simulink model "EMT_ML.before_diagnostic_fixes"  (R2024b)
settings: Solver=ode5  StartTime=0.0  StopTime=200  FixedStep=0.002  RelTol=1e-3
model workspace (MAT data in the model file):
  A = 7.3
  B = 2.71
  C0_shift = 200
  C1_shift = 200
  C2_shift = 200
  Cb = 70
  Cd = 0.6
  EMSInputBus : Simulink.Bus (value not decoded)
  Fb_max = 247500
  JA = 0.4
  JB = 0.4
  JZ = 0.4
  Jc1r2 = 0.01
  Jc3r4 = 0.01
  Jc4 = 0.01
  Je = 2.5
  Jh = 0.01
  Jq1 = 0.01
  Jq2 = 0.01
  Jr1 = 0.01
  Jr3s4 = 0.01
  Js123 = 0.01
  L = 4.472
  NE = [1600 1600 1600 1600 1600 1600 1600 1600 1600 1600 1600 1600 ... (840 elements, 30x28)]
  N_Te = 30
  N_ne = 28
  PE = [0 100.366530527 133.710336161 167.221698607 195.706356687 221.845219395 250.497434286 278.144308305 305.288511886 330.086920096 352.87464656 374.489475338 ... (840 elements, 30x28)]
  PN0 = 0
  Pb_epr = [-45 -45 -40 -30 0 30 40 45 45]
  Pb_max = [0 40 45 45 45]
  Pb_min = [-45 -45 -45 -40 0]
  Pe_ass = 230
  Pe_max = 1103
  Peg = [0 100 120 140 160 180 200 220 240 260 280 300 ... (53 elements, 1x53)]
  R_map = [0.09 0.089 0.09 0.091 0.092 0.093 0.094 0.095 0.096 0.097 0.098]
  SF_C0 = 1.5
  SF_C1 = 1.5
  SF_C2 = 1.5
  SF_Z1 = 1.5
  SF_Z2 = 1.5
  SF_ZD = 1.5
  SOC0 = 60
  SOC_epr = [30 31 50 59 60 61 70 79 80]
  SOC_map = [0 10 20 30 40 50 60 70 80 90 100]
  TA_max_map = [588.855 593.803361345 598.83559322 603.953846154 609.160344828 614.457391304 619.847368421 625.332743363 630.916071429 636.6 642.387272727 648.280733945 ... (115 elements, 1x115)]
  TA_min_map = [-588.855 -593.803361345 -598.83559322 -603.953846154 -609.160344828 -614.457391304 -619.847368421 -625.332743363 -630.916071429 -636.6 -642.387272727 -648.280733945 ... (115 elements, 1x115)]
  TAf = 0
  TB_max_map = [588.855 593.803361345 598.83559322 603.953846154 609.160344828 614.457391304 619.847368421 625.332743363 630.916071429 636.6 642.387272727 648.280733945 ... (115 elements, 1x115)]
  TB_min_map = [-588.855 -593.803361345 -598.83559322 -603.953846154 -609.160344828 -614.457391304 -619.847368421 -625.332743363 -630.916071429 -636.6 -642.387272727 -648.280733945 ... (115 elements, 1x115)]
  TBf = 0
  TE = [0 599 798 998 1168 1324 1495 1660 1822 1970 2106 2235 ... (840 elements, 30x28)]
  TS_A = 0.2
  TS_B = 0.2
  TS_C0 = 0.2
  TS_C1 = 0.2
  TS_C2 = 0.2
  TS_Z = 0.2
  TS_Z1 = 0.2
  TS_Z2 = 0.2
  TS_ZD = 0.2
  TZ_max_map = [537.13125 540.509433962 543.930379747 547.394904459 550.903846154 554.458064516 558.058441558 561.705882353 565.401315789 569.145695364 572.94 576.785234899 ... (131 elements, 1x131)]
  TZ_min_map = [-537.13125 -540.509433962 -543.930379747 -547.394904459 -550.903846154 -554.458064516 -558.058441558 -561.705882353 -565.401315789 -569.145695364 -572.94 -576.785234899 ... (131 elements, 1x131)]
  TZf = 0
  T_generator = [0 185 493.333333333 801.666666667 1110 1418.33333333 1726.66666667]
  T_motor = [0 185 493.333333333 801.666666667 1110 1418.33333333 1726.66666667]
  Te_map = [0 599 798 998 1168 1324 1495 1660 1822 1970 2106 2235 ... (30 elements, 1x30)]
  Te_max = 2754
  Te_max_map = [1168 1324 1495 1660 1822 1970 2106 2235 2355 2458 2543 2606 ... (28 elements, 1x28)]
  Te_start = 1600
  Tef = 100
  Teg = [0 596.8125 636.6 718.741935484 799.916230366 859.41 954.422788606 954.9 996.417391304 1078.98305085 1114.05 1169.26530612 ... (53 elements, 1x53)]
  Temax = 998
  Time = [0 0.1 0.2 0.3 0.4 0.5 0.6 0.7 0.8 0.9 1 1.1 ... (2001 elements, 1x2001)]
  Time_ele = [0 4 8 12 16 20 24 28 32 36 40 44 ... (401 elements, 1x401)]
  Time_fg = [0 2 4 6 8 10 12 14 16 18 20 22 ... (801 elements, 1x801)]
  Tmax_C0 = 2754
  Tmax_C1 = 3505.25455609
  Tmax_C2 = 3505.25455609
  Tmax_Z1 = 5584.80955498
  Tmax_Z2 = 16307.6439005
  Tmax_ZD = 3855.6
  Ts_e = 0.1
  Uoc_map = [814.5 917 933.25 945.75 958.25 969.25 978 985.25 993.25 1003.25 1050]
  V_Shift12 = 32
  V_Shift21 = 25
  V_Start = 10
  Voltage0 = 900
  Voltage_epr = [750 760 900 1000 1050]
  Y_engine = 0.955
  Yc = 0.98
  Yh = 0.96
  Yo = 0.92
  Yq = 0.94
  Z1_shift = 200
  Z2_shift = 200
  a11 = 1.54241568346
  a11_L = 1.54241568346
  a12 = -3.86074191629
  a12_L = 2.43173643789
  a21 = -1.04963112005
  a22 = 2.46948356808
  b11 = 0
  b11_L = 0
  b12 = 3.33
  b12_L = 7.8036
  b21 = 2.23571428571
  b22 = -2.13
  c11 = -0.648333656565
  c12 = 0
  c21 = -0.648333656565
  c22 = 0.680511182109
  controller_id = 1
  controller_name = 'Existing heuristic-grid EMS'
  cycle_grade = [0 0 0 0 0 0 0 0 0 0 0 0 ... (2001 elements, 1x2001)]
  cycle_road = [0.045 0.045 0.045 0.045 0.045 0.045 0.045 0.045 0.045 0.045 0.045 0.045 ... (2001 elements, 1x2001)]
  cycle_steering = [0 0 0 0 0 0 0 0 0 0 0 0 ... (2001 elements, 1x2001)]
  cycle_time = [0 0.1 0.2 0.3 0.4 0.5 0.6 0.7 0.8 0.9 1 1.1 ... (2001 elements, 1x2001)]
  d11 = -0.751666343435
  d12 = 0.3003003003
  d21 = -0.751666343435
  d22 = 0.319488817891
  e11 = -1.54241568346
  e12 = 0
  e21 = 1.04963112005
  e22 = -2.23571428571
  eff_generator = [0.8 0.8 0.79 0.79 0.76 0.74 0.72 0.8 0.85 0.88 0.85 0.8 ... (84 elements, 7x12)]
  eff_motor = [0.8 0.8 0.79 0.79 0.76 0.74 0.72 0.8 0.85 0.88 0.85 0.8 ... (84 elements, 7x12)]
  ele_map = [10 11.46 14.13 19.24 20.94 23.21 20.29 20.23 22.28 17.66 16.24 18.95 ... (401 elements, 1x401)]
  ems_runtime_config : object (value not decoded)
  f11 = -3.86074191629
  f12 = 3.33
  f21 = 2.46948356808
  f22 = -2.13
  fg = 0.045
  fg_map = [0.0125 0.0215 0.0332 0.0452 0.0525 0.0589 0.0584 0.0592 0.0621 0.0576 0.055 0.0572 ... (801 elements, 1x801)]
  fuel_gpkwh = [269.874826377 269.874826377 260.084605263 254.895150301 249.802821062 244.062054381 234.972466555 226.630558735 223.93243551 227.612775381 231.379615385 228.983738255 ... (840 elements, 30x28)]
  fuel_map = [269.874826377 269.874826377 260.084605263 254.895150301 249.802821062 244.062054381 234.972466555 226.630558735 223.93243551 227.612775381 231.379615385 228.983738255 ... (840 elements, 30x28)]
  fuel_map_N = [269.874826377 269.874826377 260.084605263 254.895150301 249.802821062 nan nan nan nan nan nan nan ... (840 elements, 30x28)]
  i = 28
  ic = 4.42
  iq = 1.4
  it = 4
  j = 30
  k1 = 2.13
  k2 = 2.13
  k3 = 2.33
  k4 = 1.92
  kh = 2.88
  kq = 2.17
  kt = 1.83
  mass = 45000
  miu_max = 0.8
  nA_map = [-6000 -5950 -5900 -5850 -5800 -5750 -5700 -5650 -5600 -5550 -5500 -5450 ... (115 elements, 1x115)]
  nA_max = 6000
  nA_min = -6000
  nB_map = [-6000 -5950 -5900 -5850 -5800 -5750 -5700 -5650 -5600 -5550 -5500 -5450 ... (115 elements, 1x115)]
  nB_max = 6000
  nB_min = -6000
  nB_start = 0
  nZ_map = [-8000 -7950 -7900 -7850 -7800 -7750 -7700 -7650 -7600 -7550 -7500 -7450 ... (131 elements, 1x131)]
  nZ_max = 8000
  nZ_min = -8000
  n_generator = [0 318.5 796.25 1274 1751.75 2229.5 2707.25 3185 3662.75 4140.5 4618.25 7007]
  n_motor = [0 318.5 796.25 1274 1751.75 2229.5 2707.25 3185 3662.75 4140.5 4618.25 7007]
  ne_idl = 3000
  ne_map = [1600 1700 1800 1900 2000 2100 2200 2300 2400 2500 2600 2700 ... (28 elements, 1x28)]
  ne_max = 4200
  ne_min = 1600
  ne_start = 200
  neg = [1600 1600 1800 1860 1910 2000 2001 2200 2300 2301 2400 2450 ... (53 elements, 1x53)]
  no_Shift12 = 1589.43589002
  no_Shift21 = 1241.74678908
  rz = 0.318
  startup_feedback_delay_s = 0.002
  startup_power_share = 0.5
  startup_speed_regularizer_rpm = 100
  v_cyc = [0 0 0 0 0 0 0 0 0 0 0 0 ... (2001 elements, 1x2001)]
  voltage_HighA = 1050
  voltage_HighB = 1050
  voltage_HighZ = 1050
  voltage_LowA = 750
  voltage_LowB = 750
  voltage_LowZ = 750
symbols that are objects in the model workspace (value not decoded): ems_runtime_config
undefined symbols (not defined in the file or in its folder): sigbuilder_block
libraries: fl_lib x82, nesl_utility x55, simulink x49, sdl_lib x10, simulink_need_slupdate x6, powerlib_extras x1
(part 2 of 7)

== system EMT_ML.before_diagnostic_fixes/Battery ==
  Battery : Subsystem  mask(Battery model){Cb=Cb, SOC0=SOC0, SOC_map=SOC_map, R_map=R_map, Uoc_map=Uoc_map}
      mask prompts: Cb "Capacity (Ah)"; SOC0 "Initial SOC (%)"; SOC_map "State of Charge map (%)"; R_map "Internal resistance map (oms)"; Uoc_map "Open circult voltage map(V)"
      mask help:
      | The length of Open circult voltage map and Internal resistance map is the same with State of Charge map.
      | The power of the battery is positive when it supplies energy, so it's negative when it stores energy.
  Solver Configuration : nesl_utility/Solver Configuration  PhysicalDomain=network_engine_domain  SubClassName=solver  LeftPortType=input  RightPortType=generic  Tones=[]  Harmonics=[]  SimulateNoise=off  Profile=off  UseLocalSampling=off  EnableSwitchedLinearOptims=on  FrequencyDomain=off  UseCCode=off  RelTol=0.001  AbsTol=1e-06  MinStep=1e-09  ToWorkspace=off  RevertToSquareIcSolve=off  NumHomotopyIterations=100  PhasorMode=off  PhasorModeNumHarmonics=1  ConsistencySolver=NEWTON_FTOL  IndexReductionMethod=DerivativeReplacement  DoDC=off  ResidualTolerance=1e-9  ConsistencyTolSource=GLOBAL  ConsistencyAbsTol=0.001  ConsistencyRelTol=0.001  ConsistencyTolFactor=0.001  UseLocalSolver=off  LocalSolverChoice=NE_BACKWARD_EULER_ADVANCER  ResolveIndetEquations=on  FunctionEvalNumThread=1  LocalSolverSampleTime=.001  DoFixedCost=off  MaxNonlinIter=3  MaxModeIter=2  ComputeImpulses=off  ImpulseIterations=2  LinearAlgebra=Sparse  LinearAlgebraNumThread=0  EquationFormulation=NE_TIME_EF  DelaysMemoryBudget=1024  AutomaticFiltering=on  FilteringTimeConstant=0.001  PartitionStorageMethod=AS_NEEDED  PartitionMemoryBudget=1024  PartitionMethod=FAST  MultibodyUseLocalSolver=off  MultibodyLocalSolverChoice=ODE1  MultibodyLocalSolverSampleTime=0.001
  State : Subsystem
  + bat : PMIOPort  Side=Left
  - bat : PMIOPort  Port=2  Side=Left
  wires:
  Battery/1(Voltage) -> State/1(U)
  Battery/2(Current) -> State/2(I)
  Battery/3(SOC) -> State/3(SOC)
  [ElectricPower] -> Battery/1(ElectricPower)
  connections:
  - bat/RConn1 -- Battery/LConn2 -- Solver Configuration/RConn1
  Battery/LConn1 -- + bat/RConn1

== system EMT_ML.before_diagnostic_fixes/Control Unit ==
  Control : Subsystem
  Demux : Demux  Outputs=7
      settings: DisplayOption=none
  Driver : Subsystem
  tag scope: Fb_com=global, Press=global, TA_com=global, TB_com=global, TZ_com=global, Te_com=global, engine_switch=global
  wires:
  Control/1(command) -> Demux/1
  Demux/1 -> [Press]
  Demux/2 -> [engine_switch]
  Demux/3 -> [Te_com]
  Demux/4 -> [TA_com]
  Demux/5 -> [TB_com]
  Demux/6 -> [TZ_com]
  Demux/7 -> [Fb_com]

== system EMT_ML.before_diagnostic_fixes/Front Gear ==
  C0 : Subsystem
  Subsystem : Subsystem
  iq : sdl_lib/Gears/Simple Gear  ratio=iq  rotation_direction=3-2*(1)  friction_model=2  T_noload=0.1 N*m  T_nom=5 N*m  efficiency_nom=0.8  efficiency=Yq  temperature_TLU=[ 280 300 320 ] K  load_TLU=[ 1 5 10 ] N*m  efficiency_TLU=[ 0.95 0.9 0.85 ]  efficiency_TLU2=[ 0.85 0.8 0.75; 0.95 0.9 0.85; 0.85 0.8 0.7 ]  w_thr=0.01 rad/s  pwr_thr=0.001 W  enable_backlash=false  hardstop_model=simscape.enum.hardstop.smooth  backlash_distance=1e-3 mm  r_base=0.1 m  transition=1e-4 mm  backlash_stiffness=1e6 N/m  backlash_damping=1e3 N*s/m  coeff_rest=0.7  v_tol=0.001 m/s  f_tol=0 N  mu_visc=[ 0 0 ] N*m/(rad/s)  thermal_mass=50 J/K  temperature_specify=off  temperature_priority=High  temperature=300 K  temperature_nominal_specify=off  temperature_nominal_value=1  temperature_nominal_unit=K  x_backlash_specify=off  x_backlash_priority=None  x_backlash=0 mm  x_backlash_nominal_specify=off  x_backlash_nominal_value=1  x_backlash_nominal_unit=mm  f_hardstop_specify=off  f_hardstop_priority=None  f_hardstop=0 N  f_hardstop_nominal_specify=off  f_hardstop_nominal_value=1  f_hardstop_nominal_unit=N  v_backlash_specify=off  v_backlash_priority=None  v_backlash=0 m/s  v_backlash_nominal_specify=off  v_backlash_nominal_value=1  v_backlash_nominal_unit=m/s
  In : PMIOPort  Side=Left
  Out : PMIOPort  Port=2  Side=Right
  tag scope: Pi_act=global
  wires:
  Subsystem/1(power) -> [Pi_act]
  connections:
  C0/RConn1 -- iq/LConn1
  Subsystem/RConn1 -- C0/LConn1
  In/RConn1 -- Subsystem/LConn1
  iq/RConn1 -- Out/RConn1

== system EMT_ML.before_diagnostic_fixes/Power Coupler  ==
  C1 : Subsystem
  Z1 : Subsystem
  Z2 : Subsystem
  k1 : sdl_lib/Gears/Planetary Gear  rs_ratio=k1  friction_model=2  efficiency=[ 0.97 0.98 ]  temperature_TLU=[ 280 300 320 ] K  efficiency_sp_TLU=[ 0.95 0.9 0.85 ]  efficiency_rp_TLU=[ 0.95 0.9 0.85 ]  pwr_thr=[ 0.001 0.001 ] W  mu_visc=[ 0 0 ] N*m/(rad/s)  model_inertia=0  sun_inertia=1e-10 kg*m^2  ring_inertia=1e-10 kg*m^2  carrier_inertia=1e-10 kg*m^2  carrier_radius=0.01 m  planet_inertia=0.001 kg*m^2  planet_mass=1e-10 kg  thermal_mass=50 J/K  T_init=300 K
  k2 : sdl_lib/Gears/Planetary Gear  rs_ratio=k2  friction_model=2  efficiency=[ 0.97 0.98 ]  temperature_TLU=[ 280 300 320 ] K  efficiency_sp_TLU=[ 0.95 0.9 0.85 ]  efficiency_rp_TLU=[ 0.95 0.9 0.85 ]  pwr_thr=[ 0.001 0.001 ] W  mu_visc=[ 0 0 ] N*m/(rad/s)  model_inertia=0  sun_inertia=1e-10 kg*m^2  ring_inertia=1e-10 kg*m^2  carrier_inertia=1e-10 kg*m^2  carrier_radius=0.01 m  planet_inertia=0.001 kg*m^2  planet_mass=1e-10 kg  thermal_mass=50 J/K  T_init=300 K
  k3 : sdl_lib/Gears/Planetary Gear  rs_ratio=k3  friction_model=2  efficiency=[ 0.97 0.98 ]  temperature_TLU=[ 280 300 320 ] K  efficiency_sp_TLU=[ 0.95 0.9 0.85 ]  efficiency_rp_TLU=[ 0.95 0.9 0.85 ]  pwr_thr=[ 0.001 0.001 ] W  mu_visc=[ 0 0 ] N*m/(rad/s)  model_inertia=0  sun_inertia=1e-10 kg*m^2  ring_inertia=1e-10 kg*m^2  carrier_inertia=1e-10 kg*m^2  carrier_radius=0.01 m  planet_inertia=0.001 kg*m^2  planet_mass=1e-10 kg  thermal_mass=50 J/K  T_init=300 K
  k4 : sdl_lib/Gears/Planetary Gear  rs_ratio=k4  friction_model=2  efficiency=[ 0.97 0.98 ]  temperature_TLU=[ 280 300 320 ] K  efficiency_sp_TLU=[ 0.95 0.9 0.85 ]  efficiency_rp_TLU=[ 0.95 0.9 0.85 ]  pwr_thr=[ 0.001 0.001 ] W  mu_visc=[ 0 0 ] N*m/(rad/s)  model_inertia=0  sun_inertia=1e-10 kg*m^2  ring_inertia=1e-10 kg*m^2  carrier_inertia=1e-10 kg*m^2  carrier_radius=0.01 m  planet_inertia=0.001 kg*m^2  planet_mass=1e-10 kg  thermal_mass=50 J/K  T_init=300 K
  motor A : PMIOPort  Tag=PMCPort  Side=Left
  motor B : PMIOPort  Tag=PMCPort  Port=2  Side=Right
  lnput : PMIOPort  Tag=PMCPort  Port=3  Side=Left
  output : PMIOPort  Tag=PMCPort  Port=4  Side=Right
  connections:
  k3/RConn2 -- k2/RConn2 -- k1/RConn2 -- motor B/RConn1
  C1/LConn1 -- k1/LConn1 -- k2/RConn1
  k1/RConn1 -- motor A/RConn1
  Z2/LConn1 -- k3/RConn1 -- k4/RConn2
  output/RConn1 -- k3/LConn1 -- C1/RConn1 -- k4/RConn1
  Z1/LConn1 -- k4/LConn1
  lnput/RConn1 -- k2/LConn1

== system EMT_ML.before_diagnostic_fixes/Rear Gear ==
  Rear Gear : Subsystem
  Subsystem : Subsystem
  vehicle : PMIOPort  Side=Right
  output : PMIOPort  Port=2  Side=Left
  tag scope: Po_act=global
  wires:
  Subsystem/1(power) -> [Po_act]
  connections:
  vehicle/RConn1 -- Rear Gear/RConn1
  output/RConn1 -- Subsystem/LConn1
  Subsystem/RConn1 -- Rear Gear/LConn1

== system EMT_ML.before_diagnostic_fixes/Simulation Results ==
  Battery Viewer : Subsystem
      mask Display: disp('Battery')
  Clutch & Brake Viewer : Subsystem
      mask Display: disp('Clutches && Brakes')
  Control Viewer : Subsystem
      mask Display: disp('Control')
  Engine Viewer : Subsystem
      mask Display: disp('Engine')
  Vehicle Viewer : Subsystem
      mask Display: disp('Vehicle')
  motorA Viewer : Subsystem
      mask Display: disp('Motor A')
  motorB Viewer : Subsystem
      mask Display: disp('Motor B')
  motorZ Viewer : Subsystem
      mask Display: disp('Motor Z')

== system EMT_ML.before_diagnostic_fixes/Vehicle dynamics ==
  State : Subsystem
  vehicle dynamic : Subsystem  mask{mass=mass, A=A, rz=rz, L=L, B=B, Cd=Cd, miu_max=miu_max}
      mask prompts: mass "Entire vehicle mass (kg)"; A "Windward area (m^2)"; rz "Radius of the wheel(m)"; L "Length of track (m)"; B "Width of track (m)"; Cd "Drag coefficient"; miu_max "Steering resistance coefficient"
  vehicle : PMIOPort  Side=Left
  wires:
  vehicle dynamic/2(Td_Left) -> State/2(Td_Left)
  vehicle dynamic/1(v_Left) -> State/1(v_Left)
  vehicle dynamic/4(v_Right) -> State/4(v_Right)
  vehicle dynamic/5(Td_rRght) -> State/5(Td_Right)
  [Fb_com] -> vehicle dynamic/1(Fb)
  vehicle dynamic/3(Tf_Left) -> State/3(Tf_Left)
  vehicle dynamic/6(Tf_rRght) -> State/6(Tf_Right)
  [fg_act] -> vehicle dynamic/2(fg)
  [angle] -> vehicle dynamic/3(angle)
  connections:
  vehicle/RConn1 -- vehicle dynamic/LConn1 -- vehicle dynamic/LConn2

== system EMT_ML.before_diagnostic_fixes/engine ==
  Engine : Subsystem  mask(Engine){ne_map=ne_map, Te_max_map=Te_max_map, Tef=Tef, Je=Je, T=Ts_e, Y_engine=Y_engine, P_ass=Pe_ass, Te_start=Te_start}
      mask prompts: ne_map "External characteristic speed (r/min)"; Te_max_map "External characteristic torque(Nm)"; Tef "frictional resistance (Nm)"; Je "rotational inertia(kg/m^2)"; T "First-order delay time  (s)"; Y_engine "Efficinecy of the engine"; P_ass "Power Requriement of auxiliaries (kW)"; Te_start "Engine start torque"
      mask help: Just input the parameters.
  Solver Configuration : nesl_utility/Solver Configuration  PhysicalDomain=network_engine_domain  SubClassName=solver  LeftPortType=input  RightPortType=generic  Tones=[]  Harmonics=[]  SimulateNoise=off  Profile=off  UseLocalSampling=off  EnableSwitchedLinearOptims=on  FrequencyDomain=off  UseCCode=off  RelTol=0.001  AbsTol=1e-06  MinStep=1e-09  ToWorkspace=off  RevertToSquareIcSolve=off  NumHomotopyIterations=100  PhasorMode=off  PhasorModeNumHarmonics=1  ConsistencySolver=NEWTON_FTOL  IndexReductionMethod=DerivativeReplacement  DoDC=off  ResidualTolerance=1e-9  ConsistencyTolSource=GLOBAL  ConsistencyAbsTol=0.001  ConsistencyRelTol=0.001  ConsistencyTolFactor=0.001  UseLocalSolver=off  LocalSolverChoice=NE_BACKWARD_EULER_ADVANCER  ResolveIndetEquations=on  FunctionEvalNumThread=1  LocalSolverSampleTime=.001  DoFixedCost=off  MaxNonlinIter=3  MaxModeIter=2  ComputeImpulses=off  ImpulseIterations=2  LinearAlgebra=Sparse  LinearAlgebraNumThread=0  EquationFormulation=NE_TIME_EF  DelaysMemoryBudget=1024  AutomaticFiltering=on  FilteringTimeConstant=0.001  PartitionStorageMethod=AS_NEEDED  PartitionMemoryBudget=1024  PartitionMethod=FAST  MultibodyUseLocalSolver=off  MultibodyLocalSolverChoice=ODE1  MultibodyLocalSolverSampleTime=0.001
  State : Subsystem
  Connection Port : PMIOPort  Side=Right
  wires:
  Engine/1(ne_act) -> State/1(ne)
  Engine/2(Te_act) -> State/2(Te)
  [engine_switch] -> Engine/2(switch)
  [Te_com] -> Engine/1(Te_com)
  connections:
  Connection Port/RConn1 -- Engine/RConn1 -- Solver Configuration/RConn1

== system EMT_ML.before_diagnostic_fixes/motorA ==
  Motor : Subsystem  mask(Motor){nm_map=nA_map, Tm_max_map=TA_max_map*1.5, Tm_min_map=TA_min_map*1.5, Tmf=TAf, Jm=JA, n_motor=n_motor, T_motor=T_motor, eff_motor=eff_motor, n_generator=n_generator, T_generator=T_generator, eff_generator=eff_generator, T=TS_A}
      mask prompts: nm_map "motor speed map (r/min)"; Tm_max_map "motor max torque map (Nm)"; Tm_min_map "motor min torque map  (Nm)"; Tmf "frictional resistance   (Nm)"; Jm "rotational inertia (km/m^2)"; n_motor "motor speed (r/min)"; T_motor "motor torque (Nm)"; eff_motor "motor efficiency"; n_generator "generator speed (r/min)"; T_generator "generator torque  (Nm)"; eff_generator "generator efficiency"; T "First-order delay time  (s)"
      mask help: The external and efficiency characteristics are needed. When the speed of the motor is too low or too high, it will work at its lowest or highest speed. The influence between voltage and torque is considered.
  State : Subsystem
  Connection Port : PMIOPort  Side=Right
  + mot : PMIOPort  Port=2  Side=Left
  - mot : PMIOPort  Port=3  Side=Left
  wires:
  Motor/4(power_ele) -> State/4(PA)
  Motor/3(voltage) -> State/3(UA)
  Motor/2(Tm_act) -> State/2(TA)
  Motor/1(nm_act) -> State/1(nA)
  [TA_com] -> Motor/1(Tm_com)
  connections:
  - mot/RConn1 -- Motor/LConn2
  + mot/RConn1 -- Motor/LConn1
  Connection Port/RConn1 -- Motor/RConn1

== system EMT_ML.before_diagnostic_fixes/motorB ==
  Motor : Subsystem  mask(Motor){nm_map=nB_map, Tm_max_map=TB_max_map*1.5, Tm_min_map=TB_min_map*1.5, Tmf=TBf, Jm=JB, n_motor=n_motor, T_motor=T_motor, eff_motor=eff_motor, n_generator=n_generator, T_generator=T_generator, eff_generator=eff_generator, T=TS_B}
      mask prompts: nm_map "motor speed map (r/min)"; Tm_max_map "motor max torque map (Nm)"; Tm_min_map "motor min torque map  (Nm)"; Tmf "frictional resistance   (Nm)"; Jm "rotational inertia (km/m^2)"; n_motor "motor speed (r/min)"; T_motor "motor torque (Nm)"; eff_motor "motor efficiency"; n_generator "generator speed (r/min)"; T_generator "generator torque  (Nm)"; eff_generator "generator efficiency"; T "First-order delay time  (s)"
      mask help: The external and efficiency characteristics are needed. When the speed of the motor is too low or too high, it will work at its lowest or highest speed. The influence between voltage and torque is considered.
  State : Subsystem
  Connection Port : PMIOPort  Side=Left
  + mot : PMIOPort  Port=2  Side=Right
  - mot : PMIOPort  Port=3  Side=Right
  wires:
  [TB_com] -> Motor/1(Tm_com)
  Motor/1(nm_act) -> State/1(nB)
  Motor/2(Tm_act) -> State/2(TB)
  Motor/3(voltage) -> State/3(UB)
  Motor/4(power_ele) -> State/4(PB)
  connections:
  Motor/RConn1 -- Connection Port/RConn1
  + mot/RConn1 -- Motor/LConn1
  - mot/RConn1 -- Motor/LConn2

== system EMT_ML.before_diagnostic_fixes/Battery/Battery ==
  ElectricPower : Inport
  1-D Lookup Table : Lookup_n-D  NumberOfTableDimensions=1  BreakpointsForDimension1=SOC_map  Table=Uoc_map  RndMeth=Simplest
  1-D Lookup Table1 : Lookup_n-D  NumberOfTableDimensions=1  BreakpointsForDimension1=SOC_map  Table=R_map  RndMeth=Simplest
  Add1 : Sum
  Controlled Voltage Source : fl_lib/Electrical/Electrical Sources/Controlled Voltage Source
  Current Sensor : fl_lib/Electrical/Electrical Sensors/Current Sensor
  Electrical Reference : fl_lib/Electrical/Electrical Elements/Electrical Reference
  Electronic Equipment : Subsystem
  Memory : Memory  InitialCondition=SOC0
  PS-Simulink Converter1 : nesl_utility/PS-Simulink Converter  PhysicalDomain=network_engine_domain  SubClassName=ps_output  LeftPortType=input  RightPortType=output  PseudoPeriodic=off  Frequencies=[]  VectorFormat=1-D array  Unit=A  AffineConversion=off
  PS-Simulink Converter2 : nesl_utility/PS-Simulink Converter  PhysicalDomain=network_engine_domain  SubClassName=ps_output  LeftPortType=input  RightPortType=output  PseudoPeriodic=off  Frequencies=[]  VectorFormat=1-D array  Unit=V  AffineConversion=off
  SOC Estimation : Subsystem
  Simulink-PS Converter : nesl_utility/Simulink-PS Converter  PhysicalDomain=network_engine_domain  SubClassName=ps_input  LeftPortType=input  RightPortType=output  PseudoPeriodic=off  Frequencies=[]  NoiseDistribution=none  NoiseParameters=[]  Unit=V  AffineConversion=off  FilteringAndDerivatives=filter  SimscapeFilterOrder=1  InputFilterTimeConstant=.001  UdotUserProvided=1
  Simulink-PS Converter1 : nesl_utility/Simulink-PS Converter  PhysicalDomain=network_engine_domain  SubClassName=ps_input  LeftPortType=input  RightPortType=output  PseudoPeriodic=off  Frequencies=[]  NoiseDistribution=none  NoiseParameters=[]  Unit=Ohm  AffineConversion=off  FilteringAndDerivatives=filter  SimscapeFilterOrder=1  InputFilterTimeConstant=.001  UdotUserProvided=1
  Variable Resistor : fl_lib/Electrical/Electrical Elements/Variable Resistor  Rmin=0.1 Ohm  thermalEnable=false  thermal_mass=1 J/K  i_specify=off  i_priority=None  i=0 A  i_nominal_specify=off  i_nominal_value=1  i_nominal_unit=A  v_specify=off  v_priority=None  v=0 V  v_nominal_specify=off  v_nominal_value=1  v_nominal_unit=V  T_specify=off  T_priority=None  T=300 K  T_nominal_specify=off  T_nominal_value=1  T_nominal_unit=K
  Voltage Sensor : fl_lib/Electrical/Electrical Sensors/Voltage Sensor
  pumb : Constant  Value=14
  + : PMIOPort  Side=Left
  - : PMIOPort  Port=2  Side=Left
  Voltage : Outport
  Current : Outport  Port=2
  SOC : Outport  Port=3
  wires:
  Memory/1 -> 1-D Lookup Table1/1, 1-D Lookup Table/1
  1-D Lookup Table1/1 -> Simulink-PS Converter1/1
  1-D Lookup Table/1 -> Simulink-PS Converter/1
  SOC Estimation/1(SOC) -> Memory/1, SOC/1
  PS-Simulink Converter1/1 -> SOC Estimation/1(I), Current/1
  PS-Simulink Converter2/1 -> Voltage/1
  Add1/1 -> Electronic Equipment/1(power)
  ElectricPower/1 -> Add1/2
  pumb/1 -> Add1/1
  connections:
  Simulink-PS Converter1/RConn1 -- Variable Resistor/LConn1
  Controlled Voltage Source/RConn1 -- Simulink-PS Converter/RConn1
  Current Sensor/RConn1 -- PS-Simulink Converter1/LConn1
  PS-Simulink Converter2/LConn1 -- Voltage Sensor/RConn1
  Electronic Equipment/RConn2 -- Variable Resistor/RConn1 -- Voltage Sensor/RConn2 -- -/RConn1
  Electronic Equipment/RConn1 -- +/RConn1 -- Voltage Sensor/LConn1 -- Current Sensor/RConn2
  Controlled Voltage Source/RConn2 -- Variable Resistor/LConn2 -- Electrical Reference/LConn1
  Current Sensor/LConn1 -- Controlled Voltage Source/LConn1

== system EMT_ML.before_diagnostic_fixes/Battery/State ==
  U : Inport
  I : Inport  Port=2
  SOC : Inport  Port=3
  Gain : Gain  Gain=1/1000
  Product : Product  RndMeth=Zero
  tag scope: Current=global, Pb_act=global, SOC=global, Voltage=global
  wires:
  SOC/1 -> [SOC]
  I/1 -> [Current], Product/2
  U/1 -> [Voltage], Product/1
  Gain/1 -> [Pb_act]
  Product/1 -> Gain/1

== system EMT_ML.before_diagnostic_fixes/Control Unit/Control ==
  EVT1_H Stage : Subsystem
  EVT2 Stage : Subsystem
  Multiport Switch : MultiPortSwitch  DataPortOrder=Zero-based contiguous  Inputs=4  DiagnosticForDefault=None  zeroidx=on  SaturateOnIntegerOverflow=off  InputSameDT=off
  Power Distribution : Subsystem
  Prepare Stage : Subsystem
  Shift Stage : Subsystem
  Stage Judge : Subsystem
  command : Outport
  wires:
  EVT2 Stage/1(control) -> Multiport Switch/5
  Shift Stage/1(control) -> Multiport Switch/4
  EVT1_H Stage/1(control) -> Multiport Switch/3
  Prepare Stage/1(control) -> Multiport Switch/2
  Stage Judge/1(stage) -> Multiport Switch/1
  Multiport Switch/1 -> command/1

== system EMT_ML.before_diagnostic_fixes/Control Unit/Driver ==
  Electric Power Requirement : Subsystem
      mask Display: image(imread('Electric Equiments.jpg'))
  Gears : Subsystem
      mask Display: image(imread('gears.jpg'))
  Grade Angle : Subsystem
      mask Display: image(imread('Grade.jpg'))
  Ground Resistance Coefficient : Subsystem
      mask Display: image(imread('Ground.jpg'))
  "Pedal " : Subsystem
      mask Display: image(imread('pedal.jpg'))
  Wheel Angle : Subsystem
      mask Display: image(imread('Wheel.jpg'))

== system EMT_ML.before_diagnostic_fixes/Front Gear/C0 ==
  Abs : Abs  SaturateOnIntegerOverflow=off
  Add : Sum  Inputs=+-
  C0 : Subsystem
  Power : Subsystem
  Power1 : Subsystem
  In : PMIOPort  Side=Left
  Out : PMIOPort  Port=2  Side=Right
  tag scope: C0_loss=global, C0_rela=global
  wires:
  [Press_C0] -> C0/1(Press)
  C0/1(r/min) -> [C0_rela]
  Power1/1(kW) -> Add/2
  Power/1(kW) -> Add/1
  Add/1 -> Abs/1
  Abs/1 -> [C0_loss]
  connections:
  In/RConn1 -- Power/LConn1
  C0/LConn1 -- Power/RConn1
  C0/RConn1 -- Power1/LConn1
  Power1/RConn1 -- Out/RConn1

== system EMT_ML.before_diagnostic_fixes/Front Gear/Subsystem ==
  Gain1 : Gain  Gain=1/9549
  Product3 : Product  RndMeth=Zero
  Speed Sensor : Subsystem  mask(Speed Sensor){}
      mask help: The speed unit is r/min.
  Torque Sensor : Subsystem  mask(Torque Sensor){}
      mask help: The torque unit is Nm.
  in : PMIOPort  Side=Left
  out : PMIOPort  Port=2  Side=Right
  power : Outport
  wires:
  Gain1/1 -> power/1
  Product3/1 -> Gain1/1
  Torque Sensor/1(Nm) -> Product3/2
  Speed Sensor/1(r/min) -> Product3/1
  connections:
  out/RConn1 -- Torque Sensor/RConn1
  Speed Sensor/LConn1 -- Torque Sensor/LConn1 -- in/RConn1

== system EMT_ML.before_diagnostic_fixes/Power Coupler /C1 ==
  Abs : Abs  SaturateOnIntegerOverflow=off
  Add : Sum  Inputs=+-
  C2 : Subsystem
  Power : Subsystem
  Power1 : Subsystem
  In : PMIOPort  Side=Left
  Out : PMIOPort  Port=2  Side=Right
  tag scope: C1_loss=global, C1_rela=global
  wires:
  C2/1(r/min) -> [C1_rela]
  [Press_C1] -> C2/1(Press)
  Add/1 -> Abs/1
  Abs/1 -> [C1_loss]
  Power1/1(kW) -> Add/2
  Power/1(kW) -> Add/1
  connections:
  In/RConn1 -- Power/LConn1
  Power/RConn1 -- C2/LConn1
  C2/RConn1 -- Power1/LConn1
  Power1/RConn1 -- Out/RConn1

== system EMT_ML.before_diagnostic_fixes/Power Coupler /Z1 ==
  Mechanical Rotational Reference : fl_lib/Mechanical/Rotational Elements/Mechanical Rotational Reference
  Z : Subsystem
  Z1 : PMIOPort  Side=Left
  connections:
  Mechanical Rotational Reference/LConn1 -- Z/RConn1
  Z1/RConn1 -- Z/LConn1

== system EMT_ML.before_diagnostic_fixes/Power Coupler /Z2 ==
  Mechanical Rotational Reference : fl_lib/Mechanical/Rotational Elements/Mechanical Rotational Reference
  Z : Subsystem
  Z2 : PMIOPort  Side=Left
  connections:
  Z/LConn1 -- Z2/RConn1
  Mechanical Rotational Reference/LConn1 -- Z/RConn1

== system EMT_ML.before_diagnostic_fixes/Rear Gear/Rear Gear ==
  Inertia : fl_lib/Mechanical/Rotational Elements/Inertia  inertia=Jh/2 kg*m^2  num_ports=foundation.enum.numPorts2.one  w_specify=on  w_priority=High  w=0 rad/s  w_nominal_specify=off  w_nominal_value=1  w_nominal_unit=rad/s  t_specify=off  t_priority=None  t=0 N*m  t_nominal_specify=off  t_nominal_value=1  t_nominal_unit=N*m
  Inertia1 : fl_lib/Mechanical/Rotational Elements/Inertia  inertia=Jc3r4/2 kg*m^2  num_ports=foundation.enum.numPorts2.one  w_specify=on  w_priority=High  w=0 rad/s  w_nominal_specify=off  w_nominal_value=1  w_nominal_unit=rad/s  t_specify=off  t_priority=None  t=0 N*m  t_nominal_specify=off  t_nominal_value=1  t_nominal_unit=N*m
  Simple Gear : sdl_lib/Gears/Simple Gear  ratio=ic*(1+kh)/kh  rotation_direction=3-2*(1)  friction_model=2  T_noload=0.1 N*m  T_nom=5 N*m  efficiency_nom=0.8  efficiency=Yh*Yc  temperature_TLU=[ 280 300 320 ] K  load_TLU=[ 1 5 10 ] N*m  efficiency_TLU=[ 0.95 0.9 0.85 ]  efficiency_TLU2=[ 0.85 0.8 0.75; 0.95 0.9 0.85; 0.85 0.8 0.7 ]  w_thr=0.01 rad/s  pwr_thr=0.001 W  enable_backlash=false  hardstop_model=simscape.enum.hardstop.smooth  backlash_distance=1e-3 mm  r_base=0.1 m  transition=1e-4 mm  backlash_stiffness=1e6 N/m  backlash_damping=1e3 N*s/m  coeff_rest=0.7  v_tol=0.001 m/s  f_tol=0 N  mu_visc=[ 0 0 ] N*m/(rad/s)  thermal_mass=50 J/K  temperature_specify=off  temperature_priority=High  temperature=300 K  temperature_nominal_specify=off  temperature_nominal_value=1  temperature_nominal_unit=K  x_backlash_specify=off  x_backlash_priority=None  x_backlash=0 mm  x_backlash_nominal_specify=off  x_backlash_nominal_value=1  x_backlash_nominal_unit=mm  f_hardstop_specify=off  f_hardstop_priority=None  f_hardstop=0 N  f_hardstop_nominal_specify=off  f_hardstop_nominal_value=1  f_hardstop_nominal_unit=N  v_backlash_specify=off  v_backlash_priority=None  v_backlash=0 m/s  v_backlash_nominal_specify=off  v_backlash_nominal_value=1  v_backlash_nominal_unit=m/s
  In : PMIOPort  Side=Left
  Out : PMIOPort  Port=2  Side=Right
  connections:
  Simple Gear/RConn1 -- Inertia/LConn1 -- Out/RConn1
  Simple Gear/LConn1 -- In/RConn1 -- Inertia1/LConn1

== system EMT_ML.before_diagnostic_fixes/Rear Gear/Subsystem ==
  Gain1 : Gain  Gain=1/9549
  Product3 : Product  RndMeth=Zero
  Speed Sensor : Subsystem  mask(Speed Sensor){}
      mask help: The speed unit is r/min.
  Torque Sensor : Subsystem  mask(Torque Sensor){}
      mask help: The torque unit is Nm.
  in : PMIOPort  Side=Left
  out : PMIOPort  Port=2  Side=Right
  power : Outport
  wires:
  Gain1/1 -> power/1
  Product3/1 -> Gain1/1
  Torque Sensor/1(Nm) -> Product3/2
  Speed Sensor/1(r/min) -> Product3/1
  connections:
  out/RConn1 -- Torque Sensor/RConn1
  Torque Sensor/LConn1 -- in/RConn1 -- Speed Sensor/LConn1

== system EMT_ML.before_diagnostic_fixes/Simulation Results/Battery Viewer ==
  Scope10 : Scope  NumInputPorts=4
  Scope2 : Scope  NumInputPorts=3
  wires:
  [SOC] -> Scope10/1
  [Current] -> Scope10/2
  [Voltage] -> Scope10/3
  [Pb_act] -> Scope10/4
  [PN_com] -> Scope2/1
  [PN_max] -> Scope2/2
  [PN_min] -> Scope2/3

== system EMT_ML.before_diagnostic_fixes/Simulation Results/Clutch & Brake Viewer ==
  Scope6 : Scope  NumInputPorts=4
  Scope7 : Scope  NumInputPorts=4
  Scope8 : Scope  NumInputPorts=4
  wires:
  [Z2_loss] -> Scope8/4
  [Z1_loss] -> Scope8/3
  [C1_loss] -> Scope8/2
  [C0_loss] -> Scope8/1
  [Z2_rela] -> Scope6/4
  [Z1_rela] -> Scope6/3
  [C1_rela] -> Scope6/2
  [C0_rela] -> Scope6/1
  [Press_Z2] -> Scope7/4
  [Press_Z1] -> Scope7/3
  [Press_C1] -> Scope7/2
  [Press_C0] -> Scope7/1

== system EMT_ML.before_diagnostic_fixes/Simulation Results/Control Viewer ==
  Scope{,1,3..4,7} (5 alike) : Scope
  Scope11 : Scope  NumInputPorts=4
  Scope2 : Scope  NumInputPorts=3
  wires:
  [Wheel] -> Scope11/4
  [angle] -> Scope11/3
  [ElectricPower] -> Scope11/2
  [fg_act] -> Scope11/1
  [stage] -> Scope2/1
  [Acc_pedal] -> Scope2/2
  [Dec_pedal] -> Scope2/3
  [Gear] -> Scope1/1
  [mode] -> Scope3/1
  [ZD_Gear] -> Scope/1
  [Wheel] -> Scope7/1
  [ElectricPower] -> Scope4/1

== system EMT_ML.before_diagnostic_fixes/Simulation Results/Engine Viewer ==
  "Fuel " : Subsystem
  Scope1 : Scope  NumInputPorts=4
  Scope12 : Scope  NumInputPorts=2
  Scope2 : Scope  NumInputPorts=3
  Scope4 : Scope  NumInputPorts=2
  Scope5 : Scope  NumInputPorts=2
  wires:
  "Fuel "/2(gpkWh) -> Scope12/2
  "Fuel "/1(fuel_L) -> Scope12/1
  [ne_act] -> Scope1/2
  [Te_act] -> Scope1/3
  [engine_switch] -> Scope1/1
  [Pe_act] -> Scope1/4
  [Pe_act] -> Scope4/2
  [Pe_com] -> Scope4/1
  [ne_act] -> Scope5/2
  [ne_ref] -> Scope5/1
  [Te_act] -> Scope2/3
  [Te_com] -> Scope2/2
  [Te_ref] -> Scope2/1

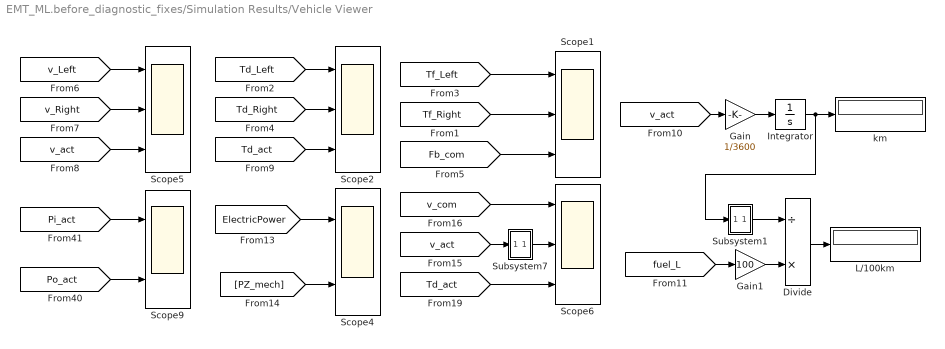
== system EMT_ML.before_diagnostic_fixes/Simulation Results/Vehicle Viewer ==
  Divide : Product  Inputs=/*
  Gain : Gain  Gain=1/3600
  Gain1 : Gain  Gain=100
  Integrator : Integrator
  L/100km : Display
  Scope{1..2,5..6} (4 alike) : Scope  NumInputPorts=3
  Scope4 : Scope  NumInputPorts=2
  Scope9 : Scope  NumInputPorts=2
  Subsystem1 : Subsystem
  Subsystem7 : Subsystem
  km : Display
  wires:
  [Pi_act] -> Scope9/1
  [Po_act] -> Scope9/2
  [v_com] -> Scope6/1
  [v_act] -> Subsystem7/1(0)
  [Td_act] -> Scope6/3
  Subsystem7/1(1) -> Scope6/2
  [v_Left] -> Scope5/1
  [v_Right] -> Scope5/2
  [v_act] -> Scope5/3
  [Td_Right] -> Scope2/2
  [Td_Left] -> Scope2/1
  [Tf_Right] -> Scope1/2
  [Tf_Left] -> Scope1/1
  [Fb_com] -> Scope1/3
  [ElectricPower] -> Scope4/1
  [PZ_mech] -> Scope4/2
  [Td_act] -> Scope2/3
  [v_act] -> Gain/1
  Integrator/1 -> km/1, Subsystem1/1(0)
  Gain/1 -> Integrator/1
  [fuel_L] -> Gain1/1
  Gain1/1 -> Divide/2
  Divide/1 -> L/100km/1
  Subsystem1/1(1) -> Divide/1

== system EMT_ML.before_diagnostic_fixes/Simulation Results/motorA Viewer ==
  Mux : Mux  Inputs=2
  Scope1 : Scope  NumInputPorts=4
  Scope2 : Scope  NumInputPorts=3
  Scope3 : Scope
  Scope4 : Scope
  wires:
  [nA_act] -> Scope1/1
  [TA_act] -> Scope1/2
  [PA_mech] -> Scope1/3
  [PA_ele] -> Scope1/4
  [PA_ele] -> Mux/2
  [PA_mech] -> Mux/1
  Mux/1 -> Scope4/1
  [voltageA] -> Scope3/1
  [TA_act] -> Scope2/3
  [TA_com] -> Scope2/2
  [TA_ref] -> Scope2/1

== system EMT_ML.before_diagnostic_fixes/Simulation Results/motorB Viewer ==
  Mux : Mux  Inputs=2
  Scope1 : Scope  NumInputPorts=4
  Scope2 : Scope  NumInputPorts=3
  Scope3 : Scope
  Scope4 : Scope
  wires:
  [PB_ele] -> Scope1/4
  [TB_act] -> Scope1/2
  [nB_act] -> Scope1/1
  [PB_mech] -> Scope1/3
  [voltageB] -> Scope3/1
  Mux/1 -> Scope4/1
  [PB_mech] -> Mux/1
  [PB_ele] -> Mux/2
  [TB_act] -> Scope2/3
  [TB_com] -> Scope2/2
  [TB_ref] -> Scope2/1

== system EMT_ML.before_diagnostic_fixes/Simulation Results/motorZ Viewer ==
  Mux : Mux  Inputs=2
  Mux1 : Mux  Inputs=2
  Scope1 : Scope  NumInputPorts=3
  Scope2 : Scope  NumInputPorts=3
  Scope3 : Scope
  Scope4 : Scope
  Scope5 : Scope  NumInputPorts=2
  Scope6 : Scope
  wires:
  [PZ_mech] -> Scope1/3
  [TZ_ref] -> Scope2/1
  [TZ_com] -> Scope2/2
  [TZ_act] -> Scope2/3
  [PZ_ele] -> Mux/2
  [PZ_mech] -> Mux/1
  Mux/1 -> Scope4/1
  [voltageZ] -> Scope3/1
  [TZ_act] -> Scope1/2
  [nZ_act] -> Scope1/1
  [nZ_ref] -> Scope5/1
  [nZ_act] -> Scope5/2
  [PZ_com] -> Mux1/2
  [PZ_ref] -> Mux1/1
  Mux1/1 -> Scope6/1

== system EMT_ML.before_diagnostic_fixes/Vehicle dynamics/State ==
  v_Left : Inport
  Td_Left : Inport  Port=2
  Tf_Left : Inport  Port=3
  v_Right : Inport  Port=4
  Td_Right : Inport  Port=5
  Tf_Right : Inport  Port=6
  Sum1 : Sum
  Sum2 : Sum
  Sum3 : Sum
  Tire Radius4 : Gain  Gain=0.5
  tag scope: Td_Left=global, Td_Right=global, Td_act=global, Tf_Left=global, Tf_Right=global, Tf_act=global, v_Left=global, v_Right=global, v_act=global
  wires:
  Td_Left/1 -> [Td_Left], Sum2/1
  v_Left/1 -> [v_Left], Sum1/1
  v_Right/1 -> [v_Right], Sum1/2
  Td_Right/1 -> [Td_Right], Sum2/2
  Sum1/1 -> Tire Radius4/1
  Sum2/1 -> [Td_act]
  Tire Radius4/1 -> [v_act]
  Tf_Left/1 -> Sum3/1, [Tf_Left]
  Tf_Right/1 -> Sum3/2, [Tf_Right]
  Sum3/1 -> [Tf_act]

== system EMT_ML.before_diagnostic_fixes/Vehicle dynamics/vehicle dynamic ==
  Fb : Inport
  fg : Inport  Port=2
  angle : Inport  Port=3
  Fb1 : InportShadow
  angle1 : InportShadow  Port=3
  fg1 : InportShadow  Port=2
  vehicle dynamic : Subsystem
  vehicle dynamic1 : Subsystem
  Left : PMIOPort  Side=Left
  Right : PMIOPort  Port=2  Side=Left
  v_Left : Outport
  Td_Left : Outport  Port=2
  Tf_Left : Outport  Port=3
  v_Right : Outport  Port=4
  Td_rRght : Outport  Port=5
  Tf_rRght : Outport  Port=6
  wires:
  Fb/1 -> vehicle dynamic/1(brake force)
  vehicle dynamic/1(vehicle speed) -> v_Left/1
  vehicle dynamic/2(Driving Torque) -> Td_Left/1
  vehicle dynamic1/1(vehicle speed) -> v_Right/1
  vehicle dynamic1/2(Driving Torque) -> Td_rRght/1
  vehicle dynamic/3(Tf) -> Tf_Left/1
  vehicle dynamic1/3(Tf) -> Tf_rRght/1
  fg/1 -> vehicle dynamic/2(fg)
  angle/1 -> vehicle dynamic/3(angle)
  Fb1/1 -> vehicle dynamic1/1(brake force)
  fg1/1 -> vehicle dynamic1/2(fg)
  angle1/1 -> vehicle dynamic1/3(angle)
  connections:
  Left/RConn1 -- vehicle dynamic/LConn1
  Right/RConn1 -- vehicle dynamic1/LConn1

== system EMT_ML.before_diagnostic_fixes/engine/Engine ==
  Te_com : Inport
  switch : Inport  Port=2
  Inertia1 : fl_lib/Mechanical/Rotational Elements/Inertia  inertia=Je kg*m^2  num_ports=foundation.enum.numPorts2.one  w_specify=on  w_priority=High  w=0 rpm  w_nominal_specify=off  w_nominal_value=1  w_nominal_unit=rad/s  t_specify=off  t_priority=None  t=0 N*m  t_nominal_specify=off  t_nominal_value=1  t_nominal_unit=N*m
  Memory2 : Memory
  Memory3 : Memory
  Speed Sensor : Subsystem  mask(Speed Sensor){}
      mask help: The speed unit is r/min.
  Subsystem : Subsystem
  Subsystem1 : Subsystem
  Torque Actuator : Subsystem  mask(Torque Actuator){}
      mask help: The torque unit is Nm.
  Out : PMIOPort  Side=Right
  ne_act : Outport
  Te_act : Outport  Port=2
  wires:
  Te_com/1 -> Subsystem/2(Te_com)
  Subsystem/2(Torque) -> Torque Actuator/1(torque)
  switch/1 -> Subsystem/3(switch)
  Memory3/1 -> Subsystem/1(ne_act)
  Speed Sensor/1(r/min) -> ne_act/1, Memory3/1, Memory2/1
  Memory2/1 -> Subsystem1/1(ne)
  Subsystem/1(Te_act) -> Te_act/1
  connections:
  Out/RConn1 -- Speed Sensor/LConn1 -- Subsystem1/RConn1 -- Torque Actuator/RConn1 -- Inertia1/LConn1

== system EMT_ML.before_diagnostic_fixes/engine/State ==
  ne : Inport
  Te : Inport  Port=2
  Gain : Gain  Gain=1/9549
  Product : Product  RndMeth=Zero
  tag scope: Pe_act=global, Te_act=global, ne_act=global
  wires:
  ne/1 -> [ne_act], Product/1
  Te/1 -> [Te_act], Product/2
  Product/1 -> Gain/1
  Gain/1 -> [Pe_act]

== system EMT_ML.before_diagnostic_fixes/motorA/Motor ==
  Tm_com : Inport
  Efficiency : Subsystem
  Electrical System : Subsystem
  Mechanical Body : Subsystem
  output : PMIOPort  Side=Right
  + mot : PMIOPort  Port=2  Side=Left
  - mot : PMIOPort  Port=3  Side=Left
  nm_act : Outport
  Tm_act : Outport  Port=2
  voltage : Outport  Port=3
  power_ele : Outport  Port=4
  wires:
  Efficiency/1(power) -> power_ele/1, Electrical System/1(power)
  Tm_com/1 -> Mechanical Body/1(Tm_com)
  Mechanical Body/2(torque) -> Efficiency/2(torque), Tm_act/1
  Mechanical Body/1(speed) -> Efficiency/1(speed), nm_act/1
  Electrical System/1(voltage) -> voltage/1
  connections:
  - mot/RConn1 -- Electrical System/RConn2
  + mot/RConn1 -- Electrical System/RConn1
  output/RConn1 -- Mechanical Body/RConn1

== system EMT_ML.before_diagnostic_fixes/motorA/State ==
  nA : Inport
  TA : Inport  Port=2
  UA : Inport  Port=3
  PA : Inport  Port=4
  Gain : Gain  Gain=1/9549
  Product : Product  RndMeth=Zero
  tag scope: PA_ele=global, PA_mech=global, TA_act=global, nA_act=global, voltageA=global
  wires:
  nA/1 -> [nA_act], Product/1
  TA/1 -> [TA_act], Product/2
  UA/1 -> [voltageA]
  PA/1 -> [PA_ele]
  Product/1 -> Gain/1
  Gain/1 -> [PA_mech]

== system EMT_ML.before_diagnostic_fixes/motorB/Motor ==
  Tm_com : Inport
  Efficiency : Subsystem
  Electrical System : Subsystem
  Mechanical Body : Subsystem
  output : PMIOPort  Side=Right
  + mot : PMIOPort  Port=2  Side=Left
  - mot : PMIOPort  Port=3  Side=Left
  nm_act : Outport
  Tm_act : Outport  Port=2
  voltage : Outport  Port=3
  power_ele : Outport  Port=4
  wires:
  Efficiency/1(power) -> power_ele/1, Electrical System/1(power)
  Tm_com/1 -> Mechanical Body/1(Tm_com)
  Mechanical Body/2(torque) -> Efficiency/2(torque), Tm_act/1
  Mechanical Body/1(speed) -> Efficiency/1(speed), nm_act/1
  Electrical System/1(voltage) -> voltage/1
  connections:
  - mot/RConn1 -- Electrical System/RConn2
  + mot/RConn1 -- Electrical System/RConn1
  output/RConn1 -- Mechanical Body/RConn1

== system EMT_ML.before_diagnostic_fixes/motorB/State ==
  nB : Inport
  TB : Inport  Port=2
  UB : Inport  Port=3
  PB : Inport  Port=4
  Gain : Gain  Gain=1/9549
  Product : Product  RndMeth=Zero
  tag scope: PB_ele=global, PB_mech=global, TB_act=global, nB_act=global, voltageB=global
  wires:
  TB/1 -> [TB_act], Product/2
  UB/1 -> [voltageB]
  PB/1 -> [PB_ele]
  Product/1 -> Gain/1
  Gain/1 -> [PB_mech]
  nB/1 -> [nB_act], Product/1

== system EMT_ML.before_diagnostic_fixes/Battery/Battery/Electronic Equipment ==
  power : Inport
  Constant3 : Constant  Value=interp1(SOC_map,Uoc_map,SOC0)
  Controlled Current Source1 : fl_lib/Electrical/Electrical Sources/Controlled Current Source
  Divie1 : Product  Inputs=*/
  Gain : Gain  Gain=-1000
  Memory2 : Memory  InitialCondition=interp1(SOC_map,Uoc_map,SOC0)
  PS-Simulink Converter : nesl_utility/PS-Simulink Converter  PhysicalDomain=network_engine_domain  SubClassName=ps_output  LeftPortType=input  RightPortType=output  PseudoPeriodic=off  Frequencies=[]  VectorFormat=1-D array  Unit=V  AffineConversion=off
  Simulink-PS Converter : nesl_utility/Simulink-PS Converter  PhysicalDomain=network_engine_domain  SubClassName=ps_input  LeftPortType=input  RightPortType=output  PseudoPeriodic=off  Frequencies=[]  NoiseDistribution=none  NoiseParameters=[]  Unit=A  AffineConversion=off  FilteringAndDerivatives=filter  SimscapeFilterOrder=1  InputFilterTimeConstant=.001  UdotUserProvided=1
  Switch : Switch  Criteria=u2 ~= 0  SaturateOnIntegerOverflow=off  InputSameDT=off
  Voltage Sensor : fl_lib/Electrical/Electrical Sensors/Voltage Sensor
  +ele : PMIOPort  Side=Right
  - ele : PMIOPort  Port=2  Side=Right
  wires:
  Gain/1 -> Simulink-PS Converter/1
  Memory2/1 -> Switch/1, Switch/2
  Switch/1 -> Divie1/2
  Constant3/1 -> Switch/3
  PS-Simulink Converter/1 -> Memory2/1
  Divie1/1 -> Gain/1
  power/1 -> Divie1/1
  connections:
  PS-Simulink Converter/LConn1 -- Voltage Sensor/RConn1
  Voltage Sensor/LConn1 -- Controlled Current Source1/LConn1 -- +ele/RConn1
  Voltage Sensor/RConn2 -- Controlled Current Source1/RConn2 -- - ele/RConn1
  Simulink-PS Converter/RConn1 -- Controlled Current Source1/RConn1

== system EMT_ML.before_diagnostic_fixes/Battery/Battery/SOC Estimation ==
  I : Inport
  Add1 : Sum
  Constant2 : Constant  Value=Cb
  Constant3 : Constant  Value=SOC0
  Divide : Product  Inputs=*/
  Gain : Gain  Gain=-1/36
  Integrator : Integrator
  SOC : Outport
  wires:
  Gain/1 -> Add1/2
  I/1 -> Divide/1
  Add1/1 -> SOC/1
  Constant3/1 -> Add1/1
  Integrator/1 -> Gain/1
  Divide/1 -> Integrator/1
  Constant2/1 -> Divide/2

== system EMT_ML.before_diagnostic_fixes/Control Unit/Control/EVT1_H Stage ==
  Mux : Mux  Inputs=7
  brack force : Subsystem
  clutches condition : Subsystem
  engine swich : Subsystem
  engine torque : Subsystem
  motorA torque : Subsystem
  motorB torque : Subsystem
  motorZ torque : Subsystem
  control : Outport
  wires:
  motorB torque/1(TB_com) -> Mux/5
  motorA torque/1(TA_com) -> Mux/4
  clutches condition/1(clutch_com) -> Mux/1
  engine swich/1(engine_swich) -> Mux/2
  engine torque/1(Te_com) -> Mux/3
  Mux/1 -> control/1
  motorZ torque/1(TZ_com) -> Mux/6
  brack force/1(Fb_com) -> Mux/7

== system EMT_ML.before_diagnostic_fixes/Control Unit/Control/EVT2 Stage ==
  Mux : Mux  Inputs=7
  brack force : Subsystem
  clutches condition : Subsystem
  engine swich : Subsystem
  engine torque : Subsystem
  motorA torque : Subsystem
  motorB torque : Subsystem
  motorZ torque : Subsystem
  control : Outport
  wires:
  motorB torque/1(TB_com) -> Mux/5
  motorA torque/1(TA_com) -> Mux/4
  engine torque/1(Te_com) -> Mux/3
  clutches condition/1(clutch_com) -> Mux/1
  engine swich/1(engine_swich) -> Mux/2
  Mux/1 -> control/1
  brack force/1(Fb_com) -> Mux/7
  motorZ torque/1(TZ_com) -> Mux/6

== system EMT_ML.before_diagnostic_fixes/Control Unit/Control/Power Distribution ==
  Electric Power Requirement : Subsystem
  Feasible Control Range : Subsystem  SystemSampleTime=0.02
  Oil Control : Subsystem
  Optimal Power Distribution : Subsystem  SystemSampleTime=10
  Pedal Interpretation : Subsystem
  Subsystem : Subsystem
  tag scope: Fb_ref=global, TA_ref=global, TB_ref=global, Te_ref=global, ne_ref=global
  wires:
  Feasible Control Range/6(TB_k) -> Optimal Power Distribution/8(TB_k)
  Feasible Control Range/5(TA_k) -> Optimal Power Distribution/7(TA_k)
  Feasible Control Range/4(Te_k) -> Optimal Power Distribution/6(Te_k)
  Feasible Control Range/3(no_k) -> Optimal Power Distribution/5(no_k)
  Feasible Control Range/2(ne_k) -> Optimal Power Distribution/4(ne_k)
  Optimal Power Distribution/1(ne_ref) -> [ne_ref]
  Electric Power Requirement/1(PN_k) -> Optimal Power Distribution/9(PN_k)
  Pedal Interpretation/2(Pe_com) -> Optimal Power Distribution/1(Pe_com)
  [stage] -> Feasible Control Range/1(stage)
  Optimal Power Distribution/4(TB_ref) -> [TB_ref]
  Optimal Power Distribution/3(TA_ref) -> [TA_ref]
  Optimal Power Distribution/2(Te_ref) -> [Te_ref]
  [v_act] -> Feasible Control Range/3(v_act)
  [ne_act] -> Feasible Control Range/2(ne_act)
  [SOC] -> Electric Power Requirement/2(SOC)
  [Voltage] -> Electric Power Requirement/1(Voltage)
  [Pedal] -> Pedal Interpretation/1(Pedal), Optimal Power Distribution/2(pedal)
  [ElectricPower] -> Electric Power Requirement/3(ElectricPower)
  Pedal Interpretation/1(Fb_ref) -> [Fb_ref]
  Feasible Control Range/1(stage_k) -> Optimal Power Distribution/3(stage_k)
  Subsystem/1(sd_ne) -> Optimal Power Distribution/10(sd_ne)

== system EMT_ML.before_diagnostic_fixes/Control Unit/Control/Prepare Stage ==
  Mux : Mux  Inputs=7
  brack force : Subsystem
  clutches condition : Subsystem
  engine swich : Subsystem
  engine torque : Subsystem
  motorA torque : Subsystem
  motorB torque : Subsystem
  motorZ torque : Subsystem
  control : Outport
  wires:
  Mux/1 -> control/1
  motorB torque/1(TB_com) -> Mux/5
  motorA torque/1(TA_com) -> Mux/4
  engine torque/1(Te_com) -> Mux/3
  engine swich/1(engine_swich) -> Mux/2
  clutches condition/1(clutch_com) -> Mux/1
  brack force/1(Fb_com) -> Mux/7
  motorZ torque/1(TZ_com) -> Mux/6

== system EMT_ML.before_diagnostic_fixes/Control Unit/Control/Shift Stage ==
  EVT1->EVT2 : Subsystem
  EVT2->EVT1 : Subsystem
  Multiport Switch : MultiPortSwitch  Inputs=2  DiagnosticForDefault=None  SaturateOnIntegerOverflow=off  InputSameDT=off
  Shift Judge : Subsystem
  control : Outport
  wires:
  Shift Judge/1(shift) -> Multiport Switch/1
  EVT2->EVT1/1(control) -> Multiport Switch/3
  EVT1->EVT2/1(control) -> Multiport Switch/2
  Multiport Switch/1 -> control/1

== system EMT_ML.before_diagnostic_fixes/Control Unit/Control/Stage Judge ==
  Add : Sum  Inputs=++++
  EVT1_H Stage : Subsystem
  EVT2 Stage : Subsystem
  Prepare Stage : Subsystem
  Shift Stage : Subsystem
  stage : Outport
  tag scope: stage=global
  wires:
  EVT2 Stage/1(Out1) -> Add/4
  EVT1_H Stage/1(Out1) -> Add/2
  Shift Stage/1(Out1) -> Add/3
  Prepare Stage/1(Out1) -> Add/1
  Add/1 -> stage/1, [stage]

== system EMT_ML.before_diagnostic_fixes/Control Unit/Driver/Electric Power Requirement ==
  " 0.1" : ManualSwitch  CurrentSetting=0
  1-D Lookup Table1 : Lookup_n-D  NumberOfTableDimensions=1  BreakpointsForDimension1=Time_ele  Table=ele_map  RndMeth=Simplest
  10 : ManualSwitch
  Add Power : ManualSwitch
  Clock1 : Clock
  ElectricPower : Display
  Saturation : Saturate  UpperLimit=300  LowerLimit=0
  Sub Power : ManualSwitch  CurrentSetting=0
  Subsystem4 : Subsystem  mask{Parameter1=on}
      mask prompts: Parameter1 "Pedal"
  Subsystem6 : Subsystem
  Transfer Fcn1 : TransferFcn  Denominator=[0.02 1]
  tag scope: ElectricPower=global
  wires:
  Subsystem4/1(Out1) -> Add Power/1
  Subsystem4/2(Out2) -> Add Power/2
  Subsystem4/3(Out3) -> Sub Power/1
  Add Power/1 -> Subsystem6/1(Add)
  Sub Power/1 -> Subsystem6/2(Sub)
  Subsystem4/4(Out4) -> Sub Power/2
  Subsystem4/5(Out5) -> " 0.1"/1
  Subsystem4/6(Out6) -> " 0.1"/2
  Subsystem4/7(Out7) -> 10/1
  Subsystem4/8(Out8) -> 10/2
  " 0.1"/1 -> Subsystem6/3(0.1)
  10/1 -> Subsystem6/4(10)
  Clock1/1 -> 1-D Lookup Table1/1
  Transfer Fcn1/1 -> [ElectricPower], ElectricPower/1
  Saturation/1 -> Transfer Fcn1/1
  1-D Lookup Table1/1 -> Saturation/1
